simulink model "abs_fuzzy_model"  (R2025a)
settings: Solver=ode4  StartTime=0.0  StopTime=10  FixedStep=0.001  RelTol=1e-3
values from neighbouring files (symbols this model uses):
  desired_slip = 0.20    (= 0.2)    [params_abs.m]
  Fr_val = Cr * m * g    (= 52.974)    [params_abs.m]
  Fz0 = m * g / 4    (= 882.9)    [params_abs.m]
  Iw = 0.5 * mw * R^2    (= 1.024)    [params_abs.m]
  K_Fa = 0.5 * rho * Cd * Af    (= 0.288372)    [params_abs.m]
  K_Fl = -m * hcg / (2 * L)    (= -32.967032967)    [params_abs.m]
  Kb = 13.0    (= 13)    [params_abs.m]
  m = 360.0    (= 360)    [params_abs.m]
  mu_table = mu_dry    [params_abs.m]
  omega0 = v0 / R    (= 52.09375)    [params_abs.m]
  P_max = 3.0e6    (= 3000000)    [params_abs.m]
  P_min = 0.0    (= 0)    [params_abs.m]
  R = 0.32    [params_abs.m]
  slip_table = [0.00, 0.05, 0.10, 0.15, 0.20, 0.25, 0.30, 0.35, 0.40, 0.50, 0.60, 0.70, 0.80, 0.90, 1.00]    [params_abs.m]
  v0 = 16.67    [params_abs.m]
  v_stop = 0.02    [params_abs.m]
libraries: fuzblock x1
settings Model: Creator=ZORO  LastModifiedBy=ZORO

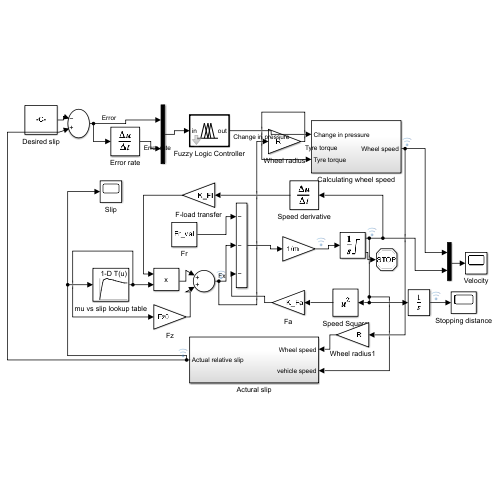
[thumbnail: Simulink's stored preview of the top-level diagram]
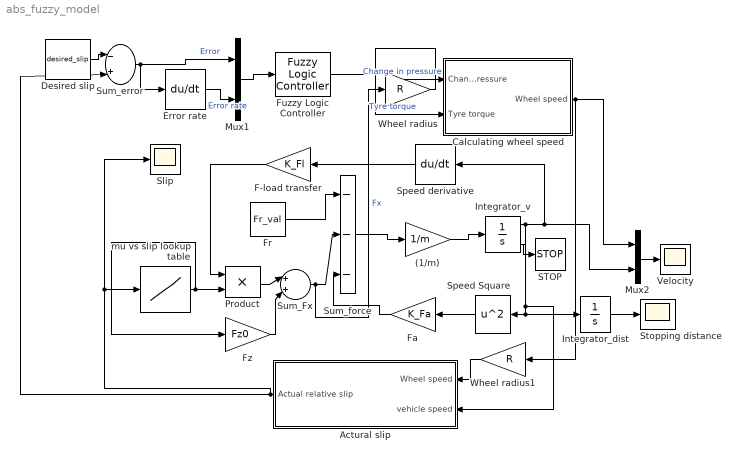
== system abs_fuzzy_model ==
  (1/m) : Gain  Gain=1/m
  Actural slip : Subsystem
  Calculating wheel speed : Subsystem
  Desired slip : Constant  Value=desired_slip
  Error rate : Derivative
  F-load transfer : Gain  Gain=K_Fl
  Fa : Gain  Gain=K_Fa
  Fr : Constant  Value=Fr_val
  Fuzzy Logic Controller : fuzblock/Fuzzy Logic  Controller  FIS='abs_fuzzy.fis'  OutputSampleNumber=101  DataType=double  UseLookupTable=off  NumBreakpoints=10  FuzzifiedInputs=off  RuleFiringStrengths=off  RuleOutputs=off  AggregatedOutputs=off  SimulateUsing=Interpreted execution  OutOfRangeInputValueMessage=none  NoRuleFiredMessage=none  EmptyOutputFuzzySetMessage=none
  Fz : Gain  Gain=Fz0
  Integrator_dist : Integrator
  Integrator_v : Integrator  InitialCondition=v0  LimitOutput=on  LowerSaturationLimit=v_stop  ShowSaturationPort=on
  Mux1 : Mux  Inputs=2
  Mux2 : Mux  Inputs=2
  Product : Product
  STOP : Stop
  Slip : Scope
  Speed Square : Math  Operator=square
  Speed derivative : Derivative
  Stopping distance : Scope
  Sum_Fx : Sum  Inputs=|++|
  Sum_error : Sum  Inputs=|-+|
  Sum_force : Sum  Inputs=---
  Velocity : Scope
  Wheel radius : Gain  Gain=R
  Wheel radius1 : Gain  Gain=R
  mu vs slip lookup table : Lookup_n-D  NumberOfTableDimensions=1  BreakpointsForDimension1=slip_table  Table=mu_table  InternalRulePriority=Speed  RndMeth=Simplest
  wires:
  Desired slip/1 -> Sum_error/1
  Sum_error/1 -> Mux1/1, Error rate/1  "Error"
  Error rate/1 -> Mux1/2  "Error rate"
  Mux1/1 -> Fuzzy Logic Controller/1
  Fuzzy Logic Controller/1 -> Calculating wheel speed/1(Change in pressure)  "Change in pressure"
  Calculating wheel speed/1(Wheel speed) -> Mux2/1, Wheel radius1/1
  Wheel radius1/1 -> Actural slip/1(Wheel speed)
  Actural slip/1(Actual relative slip) -> Slip/1, mu vs slip lookup table/1, Sum_error/2
  mu vs slip lookup table/1 -> Product/2, Fz/1
  Speed derivative/1 -> F-load transfer/1
  F-load transfer/1 -> Product/1
  Product/1 -> Sum_Fx/1
  Fz/1 -> Sum_Fx/2
  Sum_Fx/1 -> Sum_force/2, Wheel radius/1  "Fx"
  Wheel radius/1 -> Calculating wheel speed/2(Tyre torque)  "Tyre torque"
  Fr/1 -> Sum_force/1
  Speed Square/1 -> Fa/1
  Fa/1 -> Sum_force/3
  Sum_force/1 -> (1/m)/1
  (1/m)/1 -> Integrator_v/1
  Integrator_v/1 -> Integrator_dist/1, Speed Square/1, Actural slip/2(vehicle speed), Speed derivative/1, Mux2/2
  Integrator_v/2 -> STOP/1
  Mux2/1 -> Velocity/1
  Integrator_dist/1 -> Stopping distance/1

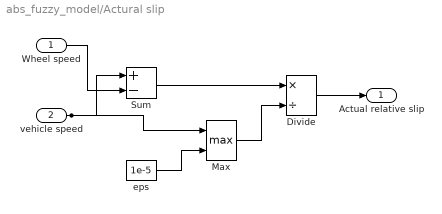
== system abs_fuzzy_model/Actural slip ==
  Wheel speed : Inport
  vehicle speed : Inport  Port=2
  Divide : Product  Inputs=*/
  Max : MinMax  Function=max  Inputs=2
  Sum : Sum  Inputs=+-
  eps : Constant  Value=1e-5
  Actual relative slip : Outport
  wires:
  vehicle speed/1 -> Sum/1, Max/1
  Wheel speed/1 -> Sum/2
  eps/1 -> Max/2
  Sum/1 -> Divide/1
  Max/1 -> Divide/2
  Divide/1 -> Actual relative slip/1

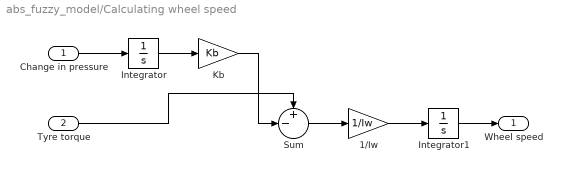
== system abs_fuzzy_model/Calculating wheel speed ==
  Change in pressure : Inport
  Tyre torque : Inport  Port=2
  1/Iw : Gain  Gain=1/Iw
  Integrator : Integrator  LimitOutput=on  UpperSaturationLimit=P_max  LowerSaturationLimit=P_min
  Integrator1 : Integrator  InitialCondition=omega0  LimitOutput=on  LowerSaturationLimit=0
  Kb : Gain  Gain=Kb
  Sum : Sum  Inputs=+-|
  Wheel speed : Outport
  wires:
  Change in pressure/1 -> Integrator/1
  Integrator/1 -> Kb/1
  Kb/1 -> Sum/2
  Tyre torque/1 -> Sum/1
  Sum/1 -> 1/Iw/1
  1/Iw/1 -> Integrator1/1
  Integrator1/1 -> Wheel speed/1
